simulink model "vla_dts"  (R2019a)
settings: Solver=VariableStepAuto  StartTime=0.0  StopTime=10.0  RelTol=1e-3
libraries: xbsIndex_r4 x8
settings Model: Creator=qwerty40  LastModifiedBy=jackh
settings DataIOCC: ReturnWorkspaceOutputs=off
settings DebuggingCC: ArithmeticOperatorsInVariantConditions=warning
settings SFSimCC: SimUseLocalCustomCode=off
settings RTWCC: RTWUseLocalCustomCode=off
settings CodeAppCC: StateflowObjectComments=on

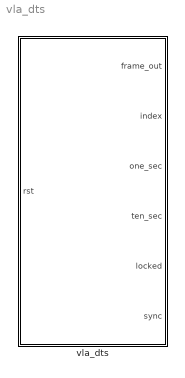
== system vla_dts ==
  vla_dts : Subsystem  Tag=xps:vla_dts  mask(vla_dts){port=qsfp_a_b_c, is_master=on, mux_factor_bits=2}
      mask prompts: port "Which port(s)?"; is_master "Is clocking master (only set this for one DTS block)"; mux_factor_bits "Multiplex factor (2^?)"
      mask help: Receive VLA DTS data
      mask init:
      | vla_dts_mask(gcb)
      mask TypeOptions port: qsfp_a_b_c | firefly0 | firefly1

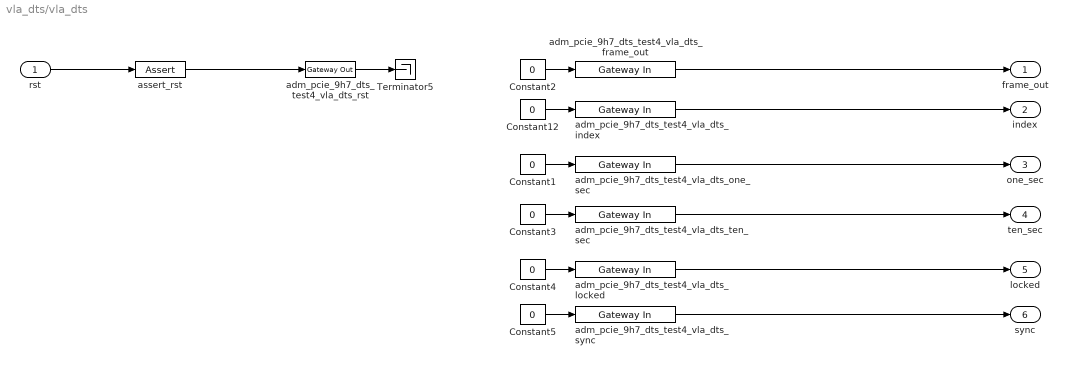
== system vla_dts/vla_dts ==
  rst : Inport
  Constant{1..5,12} (6 alike) : Constant  Value=0
  Terminator5 : Terminator
  adm_pcie_9h7_dts_test4_vla_dts_frame_out : xbsIndex_r4/Gateway In  gui_display_data_type=Fixed-point  arith_type=Unsigned  n_bits=(12*128) / (2^mux_factor_bits)  bin_pt=0  preci_type=Single  exp_width=8  frac_width=24  rows=1  columns=1  quantization=Truncate  overflow=Wrap  period=1  UseAsADC=off  ADCChannel='1'  interface=None  automatic_assignment=on  address_offset=hex2dec('00')  intf_name=''  intf_description=''  default_value=0  timing_constraint=None  locs_specified=off  LOCs={}  io_standard={}  inherit_from_input=off  hdl_port=on  dbl_ovrd=off  block_type=gatewayin
      settings: xl_area=[0, 0, 0, 0, 0, 0, 0]
  adm_pcie_9h7_dts_test4_vla_dts_index : xbsIndex_r4/Gateway In  gui_display_data_type=Fixed-point  arith_type=Unsigned  n_bits=12  bin_pt=0  preci_type=Single  exp_width=8  frac_width=24  rows=1  columns=1  quantization=Truncate  overflow=Wrap  period=1  UseAsADC=off  ADCChannel='1'  interface=None  automatic_assignment=on  address_offset=hex2dec('00')  intf_name=''  intf_description=''  default_value=0  timing_constraint=None  locs_specified=off  LOCs={}  io_standard={}  inherit_from_input=off  hdl_port=on  dbl_ovrd=off  block_type=gatewayin
      settings: xl_area=[0, 0, 0, 0, 0, 0, 0]
  adm_pcie_9h7_dts_test4_vla_dts_locked : xbsIndex_r4/Gateway In  gui_display_data_type=Fixed-point  arith_type=Unsigned  n_bits=12  bin_pt=0  preci_type=Single  exp_width=8  frac_width=24  rows=1  columns=1  quantization=Truncate  overflow=Wrap  period=1  UseAsADC=off  ADCChannel='1'  interface=None  automatic_assignment=on  address_offset=hex2dec('00')  intf_name=''  intf_description=''  default_value=0  timing_constraint=None  locs_specified=off  LOCs={}  io_standard={}  inherit_from_input=off  hdl_port=on  dbl_ovrd=off  block_type=gatewayin
      settings: xl_area=[0, 0, 0, 0, 0, 0, 0]
  adm_pcie_9h7_dts_test4_vla_dts_one_sec : xbsIndex_r4/Gateway In  gui_display_data_type=Fixed-point  arith_type=Unsigned  n_bits=12  bin_pt=0  preci_type=Single  exp_width=8  frac_width=24  rows=1  columns=1  quantization=Truncate  overflow=Wrap  period=1  UseAsADC=off  ADCChannel='1'  interface=None  automatic_assignment=on  address_offset=hex2dec('00')  intf_name=''  intf_description=''  default_value=0  timing_constraint=None  locs_specified=off  LOCs={}  io_standard={}  inherit_from_input=off  hdl_port=on  dbl_ovrd=off  block_type=gatewayin
      settings: xl_area=[0, 0, 0, 0, 0, 0, 0]
  adm_pcie_9h7_dts_test4_vla_dts_rst : xbsIndex_r4/Gateway Out  inherit_from_input=off  hdl_port=on  rows=1  columns=1  UseAsDAC=off  DACChannel='1'  interface=None  automatic_assignment=on  address_offset=hex2dec('00')  intf_name=''  intf_description=''  timing_constraint=None  locs_specified=off  LOCs={}  io_standard={}  block_type=gatewayout
      settings: infoedit="Gateway out block.  Converts Xilinx fixed point inputs into ouputs of type Simulink integer, double, or fixed point.<P><P>Hardware notes:  In hardware these blocks become top level output ports or are discarded, depending on how they are configured."  xl_area=[0, 0, 0, 0, 0, 0, 0]
  adm_pcie_9h7_dts_test4_vla_dts_sync : xbsIndex_r4/Gateway In  gui_display_data_type=Fixed-point  arith_type=Unsigned  n_bits=12  bin_pt=0  preci_type=Single  exp_width=8  frac_width=24  rows=1  columns=1  quantization=Truncate  overflow=Wrap  period=1  UseAsADC=off  ADCChannel='1'  interface=None  automatic_assignment=on  address_offset=hex2dec('00')  intf_name=''  intf_description=''  default_value=0  timing_constraint=None  locs_specified=off  LOCs={}  io_standard={}  inherit_from_input=off  hdl_port=on  dbl_ovrd=off  block_type=gatewayin
      settings: xl_area=[0, 0, 0, 0, 0, 0, 0]
  adm_pcie_9h7_dts_test4_vla_dts_ten_sec : xbsIndex_r4/Gateway In  gui_display_data_type=Fixed-point  arith_type=Unsigned  n_bits=12  bin_pt=0  preci_type=Single  exp_width=8  frac_width=24  rows=1  columns=1  quantization=Truncate  overflow=Wrap  period=1  UseAsADC=off  ADCChannel='1'  interface=None  automatic_assignment=on  address_offset=hex2dec('00')  intf_name=''  intf_description=''  default_value=0  timing_constraint=None  locs_specified=off  LOCs={}  io_standard={}  inherit_from_input=off  hdl_port=on  dbl_ovrd=off  block_type=gatewayin
      settings: xl_area=[0, 0, 0, 0, 0, 0, 0]
  assert_rst : xbsIndex_r4/Assert  assert_type=on  type_source=Explicitly  gui_display_data_type=Boolean  arith_type=Boolean  n_bits=16  bin_pt=14  preci_type=Single  exp_width=8  frac_width=24  assert_rate=on  rate_source=Explicitly  period=1  output_port=on  block_type=assert
  frame_out : Outport
  index : Outport  Port=2
  one_sec : Outport  Port=3
  ten_sec : Outport  Port=4
  locked : Outport  Port=5
  sync : Outport  Port=6
  wires:
  Constant12/1 -> adm_pcie_9h7_dts_test4_vla_dts_index/1
  Constant2/1 -> adm_pcie_9h7_dts_test4_vla_dts_frame_out/1
  rst/1 -> assert_rst/1
  assert_rst/1 -> adm_pcie_9h7_dts_test4_vla_dts_rst/1
  adm_pcie_9h7_dts_test4_vla_dts_rst/1 -> Terminator5/1
  adm_pcie_9h7_dts_test4_vla_dts_frame_out/1 -> frame_out/1
  adm_pcie_9h7_dts_test4_vla_dts_index/1 -> index/1
  adm_pcie_9h7_dts_test4_vla_dts_one_sec/1 -> one_sec/1
  Constant1/1 -> adm_pcie_9h7_dts_test4_vla_dts_one_sec/1
  Constant3/1 -> adm_pcie_9h7_dts_test4_vla_dts_ten_sec/1
  adm_pcie_9h7_dts_test4_vla_dts_ten_sec/1 -> ten_sec/1
  adm_pcie_9h7_dts_test4_vla_dts_locked/1 -> locked/1
  Constant4/1 -> adm_pcie_9h7_dts_test4_vla_dts_locked/1
  Constant5/1 -> adm_pcie_9h7_dts_test4_vla_dts_sync/1
  adm_pcie_9h7_dts_test4_vla_dts_sync/1 -> sync/1
